simulink model "VITESSE"  (R2015a)
settings: Solver=ode5  StartTime=0.0  StopTime=10.0  FixedStep=1e-3  RelTol=1e-3
libraries: simulink x1
settings Model: Creator=flapacco  LastModifiedBy=flapacco
settings DataIOCC: LimitDataPoints=off  SignalLoggingSaveFormat=ModelDataLogs  TimeSaveName=temps
settings DebuggingCC: SaveWithParameterizedLinksMsg=none  UnderspecifiedInitializationDetection=Classic  MergeDetectMultiDrivingBlocksExec=none  SolverPrmCheckMsg=warning  FcnCallInpInsideContextMsg=EnableAllAsWarning
settings HardwareCC: TargetHWDeviceType=32-bit Generic
settings GRTTargetCC: TargetFcnLib=ansi_tfl_tmw.mat  CombineOutputUpdateFcns=off  GRTInterface=on

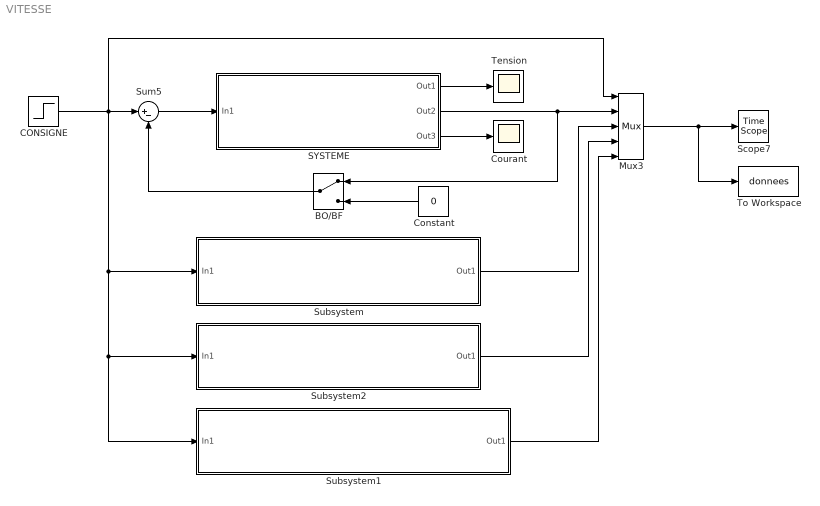
== system VITESSE ==
  BO/BF : ManualSwitch
  CONSIGNE : Step  Time=0  SampleTime=0
  Constant : Constant  Value=0
  Courant : Scope
  Mux3 : Mux  Inputs=5
  SYSTEME : Subsystem  mask(Régulation){C=0, ti=0, R=0, L=0, J=0, Jext=0, f=0, fs=0, ke=0, kt=0, UMAX=0, IMAX=0}
      mask prompts: C "Gain proportionnel C"; ti "Constante d'intégration taui (s)"; R "Résistance d'induit R (Ohms)"; L "Inductance d'induit L (H)"; J "Inertie ramenée sur l'axe moteur J (kg.m²)"; Jext "Inertie de la charge Jext (kg.m²)"; f "Frottements sur l'axe moteur f (Nm.s/rad)"; fs "Frottements secs fs (Nm)"; ke "Constante de vitesse Ke (V.s/rad)"; kt "Constante de couple Kt (Nm/A)"; UMAX "Tension maximale d'induit Umax (V)"; IMAX "Courant maximal d'induit Imax (A)"
      mask help: Régulation de niveau par correction proportionnelle
      mask init:
      | %set_param(gcb,'MaskValues',{'1','1','0.5','3','0','9.81'})
      mask Display:
      | disp('Régulateur de vitesse')
      | port_label('input',1,'Erreur')
      | port_label('output',1,'Tension induit')
      | port_label('output',2,'Vitesse')
      | port_label('output',3,'Courant induit')
  Scope7 : TimeScope
  Subsystem : Subsystem  mask{K=0, tau=0}
      mask prompts: K "Gain statique K"; tau "Constante de temps tau"
      mask Display: disp('Modèle identifié type premier ordre')
  Subsystem1 : Subsystem  mask{C=0, K=0, tau1=0, tau2=0}
      mask prompts: C "Gain proportionnel C"; K "Gain statique K"; tau1 "Constante de temps tau1"; tau2 "Constante de temps tau2"
      mask Display: disp('Modèle identifié en boucle fermée à deux constante de temps')
  Subsystem2 : Subsystem  mask{K=0, xi=0, w0=1}
      mask prompts: K "Gain statique K"; xi "Amortissement xi"; w0 "Pulsation propre w0"
      mask Display: disp('Modèle identifié type deuxième ordre')
  Sum5 : Sum  Inputs=|+-
  Tension : Scope
  To Workspace : ToWorkspace  VariableName=donnees  SampleTime=-1
  wires:
  Sum5/1 -> SYSTEME/1(In1)
  Mux3/1 -> Scope7/1, To Workspace/1
  CONSIGNE/1 -> Subsystem1/1(In1), Subsystem2/1(In1), Subsystem/1(In1), Sum5/1, Mux3/1
  SYSTEME/1(Out1) -> Tension/1
  SYSTEME/2(Out2) -> BO/BF/1, Mux3/2
  Subsystem/1(Out1) -> Mux3/3
  Subsystem2/1(Out1) -> Mux3/4
  Subsystem1/1(Out1) -> Mux3/5
  SYSTEME/3(Out3) -> Courant/1
  BO/BF/1 -> Sum5/2
  Constant/1 -> BO/BF/2

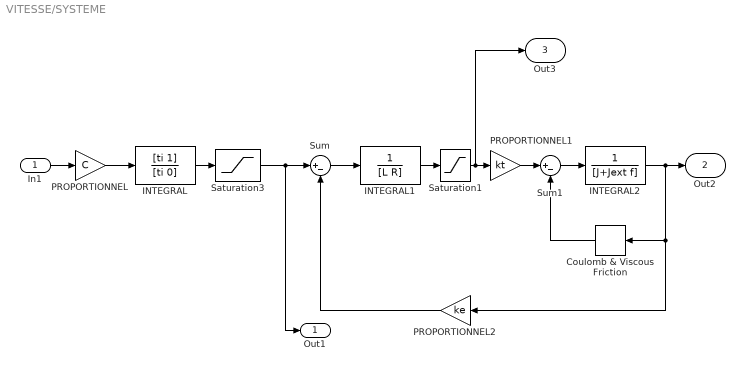
== system VITESSE/SYSTEME ==
  In1 : Inport
  Coulomb & Viscous Friction : simulink/Discontinuities/Coulomb & Viscous Friction  offset=[fs]  gain=0
  INTEGRAL : TransferFcn  Numerator=[ti 1]  Denominator=[ti 0]
  INTEGRAL1 : TransferFcn  Denominator=[L R]
  INTEGRAL2 : TransferFcn  Denominator=[J+Jext f]
  PROPORTIONNEL : Gain  Gain=C
  PROPORTIONNEL1 : Gain  Gain=kt
  PROPORTIONNEL2 : Gain  Gain=ke
  Saturation1 : Saturate  UpperLimit=IMAX  LowerLimit=-IMAX
  Saturation3 : Saturate  UpperLimit=UMAX  LowerLimit=-UMAX
  Sum : Sum  Inputs=|+-
  Sum1 : Sum  Inputs=|+-
  Out1 : Outport
  Out2 : Outport  Port=2
  Out3 : Outport  Port=3
  wires:
  Saturation3/1 -> Out1/1, Sum/1
  In1/1 -> PROPORTIONNEL/1
  PROPORTIONNEL/1 -> INTEGRAL/1
  INTEGRAL/1 -> Saturation3/1
  INTEGRAL1/1 -> Saturation1/1
  INTEGRAL2/1 -> Out2/1, PROPORTIONNEL2/1, Coulomb & Viscous Friction/1
  Sum/1 -> INTEGRAL1/1
  PROPORTIONNEL2/1 -> Sum/2
  Saturation1/1 -> PROPORTIONNEL1/1, Out3/1
  Sum1/1 -> INTEGRAL2/1
  PROPORTIONNEL1/1 -> Sum1/1
  Coulomb & Viscous Friction/1 -> Sum1/2

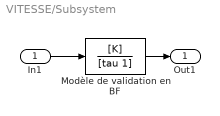
== system VITESSE/Subsystem ==
  In1 : Inport
  Modèle de validation en BF : TransferFcn  Numerator=[K]  Denominator=[tau 1]
  Out1 : Outport
  wires:
  In1/1 -> Modèle de validation en BF/1
  Modèle de validation en BF/1 -> Out1/1

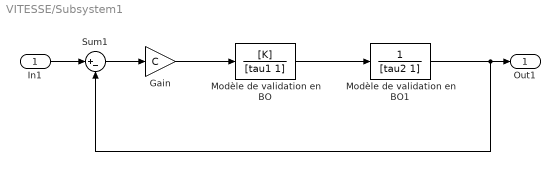
== system VITESSE/Subsystem1 ==
  In1 : Inport
  Gain : Gain  Gain=C
  Modèle de validation en BO : TransferFcn  Numerator=[K]  Denominator=[tau1 1]
  Modèle de validation en BO1 : TransferFcn  Denominator=[tau2 1]
  Sum1 : Sum  Inputs=|+-
  Out1 : Outport
  wires:
  Sum1/1 -> Gain/1
  Gain/1 -> Modèle de validation en BO/1
  Modèle de validation en BO/1 -> Modèle de validation en BO1/1
  In1/1 -> Sum1/1
  Modèle de validation en BO1/1 -> Sum1/2, Out1/1

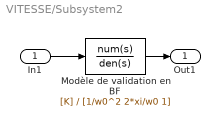
== system VITESSE/Subsystem2 ==
  In1 : Inport
  Modèle de validation en BF : TransferFcn  Numerator=[K]  Denominator=[1/w0^2 2*xi/w0 1]
  Out1 : Outport
  wires:
  In1/1 -> Modèle de validation en BF/1
  Modèle de validation en BF/1 -> Out1/1
